simulink model "hrg_wa_envelope"  (R2025a)
settings: Solver=ode4  StartTime=0.0  StopTime=wa_duration  FixedStep=wa_Ts  RelTol=1e-3
PostLoadFcn:
  | addpath(fileparts(get_param('hrg_wa_envelope','FileName'))); wa_setup;
undefined symbols (not defined in the file or in its folder): wa_controller, wa_measure, wa_nav_step, wa_p, wa_plant_rhs, wa_Ts, wa_z0
settings Model: Creator=11725  LastModifiedBy=11725
settings DataIOCC: SaveOutput=off

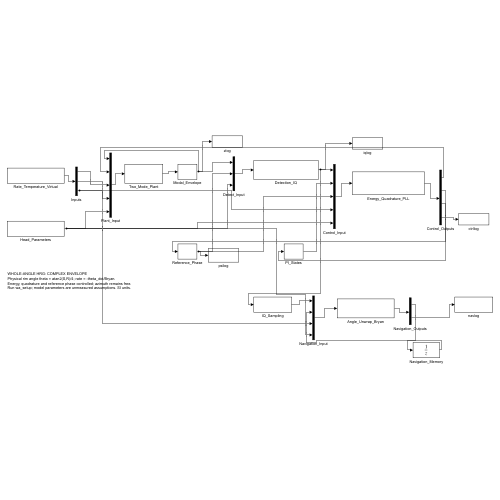
[thumbnail: Simulink's stored preview of the top-level diagram]
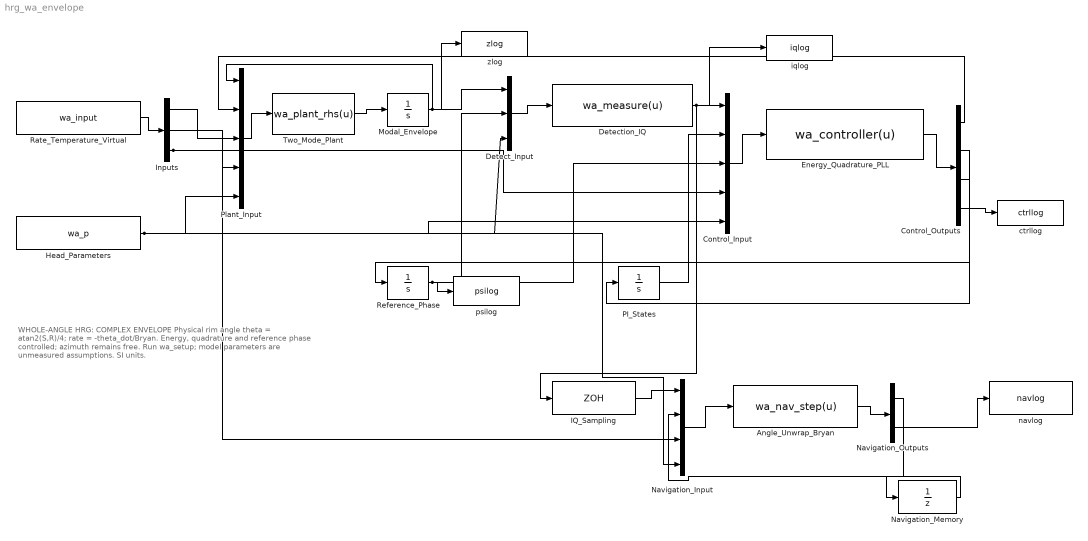
== system hrg_wa_envelope ==
  note: WHOLE-ANGLE HRG: COMPLEX ENVELOPE
      | Physical rim angle theta = atan2(S,R)/4; rate = -theta_dot/Bryan.
      | Energy, quadrature and reference phase controlled; azimuth remains free.
      | Run wa_setup; model parameters are unmeasured assumptions. SI units.
  Angle_Unwrap_Bryan : MATLABFcn  MATLABFcn=wa_nav_step(u)  OutputDimensions=8
  Control_Input : Mux  Inputs=5
  Control_Outputs : Demux  Outputs=[4 3 1 3]
  Detect_Input : Mux  Inputs=3
  Detection_IQ : MATLABFcn  MATLABFcn=wa_measure(u)  OutputDimensions=10
  Energy_Quadrature_PLL : MATLABFcn  MATLABFcn=wa_controller(u)  OutputDimensions=11
  Head_Parameters : Constant  Value=wa_p
  IQ_Sampling : ZeroOrderHold  SampleTime=wa_Ts
  Inputs : Demux  Outputs=[1 1 1]
  Modal_Envelope : Integrator  InitialCondition=wa_z0
  Navigation_Input : Mux
  Navigation_Memory : UnitDelay  InitialCondition=[0;0;0;0]  SampleTime=wa_Ts  HasFrameUpgradeWarning=on
  Navigation_Outputs : Demux  Outputs=[4 4]
  PI_States : Integrator  InitialCondition=[0;0;0]
  Plant_Input : Mux  Inputs=5
  Rate_Temperature_Virtual : FromWorkspace  VariableName=wa_input
  Reference_Phase : Integrator
  Two_Mode_Plant : MATLABFcn  MATLABFcn=wa_plant_rhs(u)  OutputDimensions=4
  ctrllog : ToWorkspace  VariableName=ctrllog  SaveFormat=Timeseries  SampleTime=-1
  iqlog : ToWorkspace  VariableName=iqlog  SaveFormat=Timeseries  SampleTime=-1
  navlog : ToWorkspace  VariableName=navlog  SaveFormat=Timeseries  SampleTime=-1
  psilog : ToWorkspace  VariableName=psilog  SaveFormat=Timeseries  SampleTime=-1
  zlog : ToWorkspace  VariableName=zlog  SaveFormat=Timeseries  SampleTime=-1
  wires:
  Modal_Envelope/1 -> Detect_Input/1, Plant_Input/1, zlog/1
  Reference_Phase/1 -> Detect_Input/2, Control_Input/3, psilog/1
  Head_Parameters/1 -> Detect_Input/3, Control_Input/5, Plant_Input/5, Navigation_Input/4
  Detect_Input/1 -> Detection_IQ/1
  Detection_IQ/1 -> Control_Input/1, IQ_Sampling/1, iqlog/1
  PI_States/1 -> Control_Input/2
  Inputs/3 -> Control_Input/4, Navigation_Input/3
  Control_Input/1 -> Energy_Quadrature_PLL/1
  Energy_Quadrature_PLL/1 -> Control_Outputs/1
  Control_Outputs/2 -> PI_States/1
  Control_Outputs/3 -> Reference_Phase/1
  Control_Outputs/1 -> Plant_Input/2
  Inputs/1 -> Plant_Input/3
  Inputs/2 -> Plant_Input/4
  Plant_Input/1 -> Two_Mode_Plant/1
  Two_Mode_Plant/1 -> Modal_Envelope/1
  Rate_Temperature_Virtual/1 -> Inputs/1
  IQ_Sampling/1 -> Navigation_Input/1
  Navigation_Memory/1 -> Navigation_Input/2
  Navigation_Input/1 -> Angle_Unwrap_Bryan/1
  Angle_Unwrap_Bryan/1 -> Navigation_Outputs/1
  Navigation_Outputs/1 -> Navigation_Memory/1
  Control_Outputs/4 -> ctrllog/1
  Navigation_Outputs/2 -> navlog/1
